simulink model "Demo_newformula"  (R2024b)
settings: Solver=FixedStepAuto  StartTime=0.0  StopTime=100  FixedStep=0.1  RelTol=1e-3
undefined symbols (not defined in the file or in its folder): LF
libraries: instrumentseriallib x4
settings Model: Creator=ihtis  LastModifiedBy=ihtisham

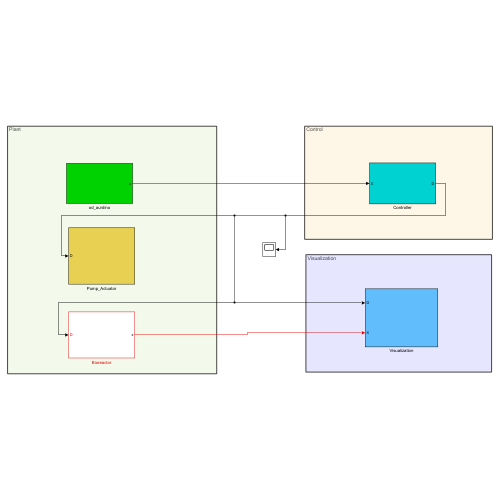
[thumbnail: Simulink's stored preview of the top-level diagram]
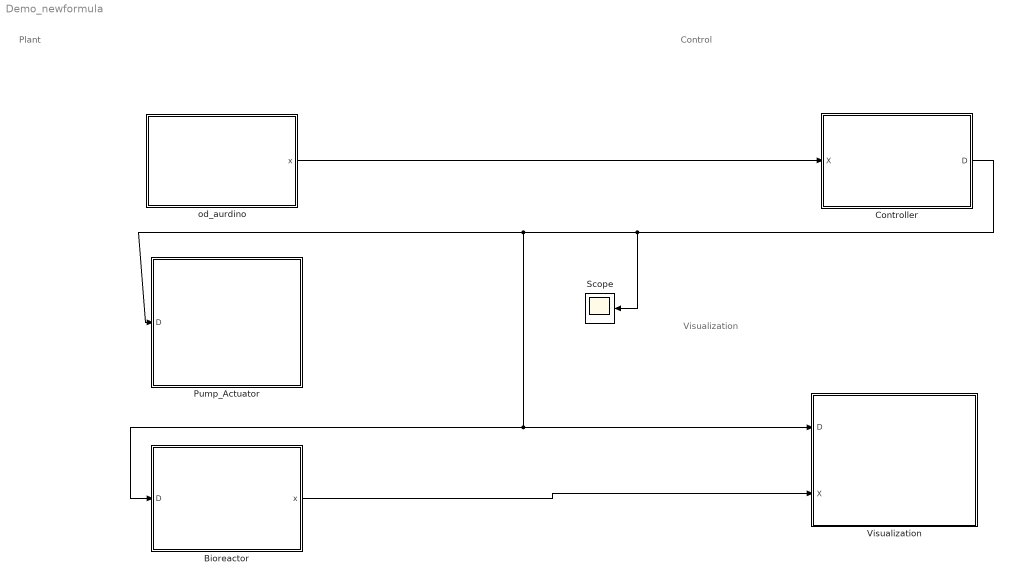
== system Demo_newformula ==
  note: Control
  note: Plant
  note: Visualization
  Bioreactor : Subsystem
  Controller : Subsystem
  Pump_Actuator : Subsystem
  Scope : Scope
  Visualization : Subsystem
  od_aurdino : Subsystem
  wires:
  Bioreactor/1(x) -> Visualization/2(X)
  Controller/1(D) -> Visualization/1(D), Bioreactor/1(D), Pump_Actuator/1(D), Scope/1
  od_aurdino/1(x) -> Controller/1(X)

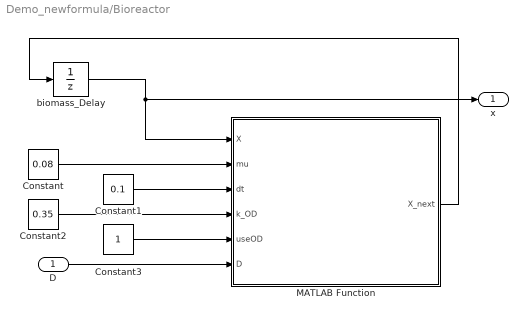
== system Demo_newformula/Bioreactor ==
  D : Inport
  Constant : Constant  Value=0.08
  Constant1 : Constant  Value=0.1
  Constant2 : Constant  Value=0.35
  Constant3 : Constant
  MATLAB Function : MATLAB Function  TreatAsAtomicUnit=on
  biomass_Delay : UnitDelay  InitialCondition=0.5  SampleTime=-1  HasFrameUpgradeWarning=on
  x : Outport
  wires:
  MATLAB Function/1(X_next) -> biomass_Delay/1
  Constant/1 -> MATLAB Function/2(mu)
  Constant1/1 -> MATLAB Function/3(dt)
  biomass_Delay/1 -> x/1, MATLAB Function/1(X)
  Constant2/1 -> MATLAB Function/4(k_OD)
  D/1 -> MATLAB Function/6(D)
  Constant3/1 -> MATLAB Function/5(useOD)

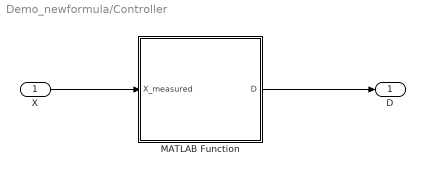
== system Demo_newformula/Controller ==
  X : Inport
  MATLAB Function : MATLAB Function  TreatAsAtomicUnit=on
  D : Outport
  wires:
  X/1 -> MATLAB Function/1(X_measured)
  MATLAB Function/1(D) -> D/1

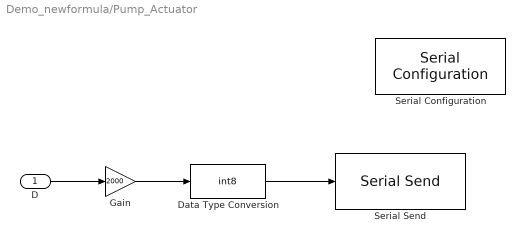
== system Demo_newformula/Pump_Actuator ==
  D : Inport
  Data Type Conversion : DataTypeConversion  OutDataTypeStr=int8  SaturateOnIntegerOverflow=off  RndMeth=Floor
  Gain : Gain  Gain=2000
  Serial Configuration : instrumentseriallib/Serial Configuration  Priority=-200000  PortSel=COM8  Port=COM8  ComPort=COM8  BaudRate=9600  DataBits=8  Parity=none  StopBits=1  ByteOrder=little-endian  FlowControl=none  Timeout=10  SimulateUsing=Interpreted execution  BlockInModel=on  aMode=1
      settings: LibrarySourceBlock=c2000lib/Host Communication/Serial Configuration
  Serial Send : instrumentseriallib/Serial Send  Priority=1  PortSel=COM8  Port=COM8  ComPort=COM8  Header=[]  Terminator=<none>  CustomTerminator=[]  EnableBlockingMode=on  SimulateUsing=Interpreted execution  BlockInModel=on  aMode=1
      settings: LibrarySourceBlock=c2000lib/Host Communication/Serial Send
  wires:
  D/1 -> Gain/1
  Gain/1 -> Data Type Conversion/1
  Data Type Conversion/1 -> Serial Send/1

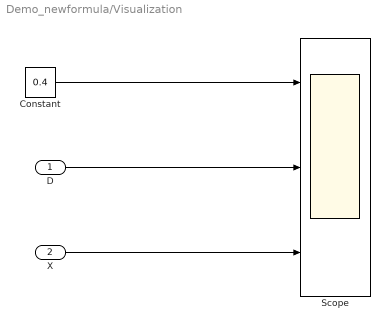
== system Demo_newformula/Visualization ==
  D : Inport
  X : Inport  Port=2
  Constant : Constant  Value=0.4
  Scope : Scope  NumInputPorts=3
  wires:
  X/1 -> Scope/3
  D/1 -> Scope/2
  Constant/1 -> Scope/1

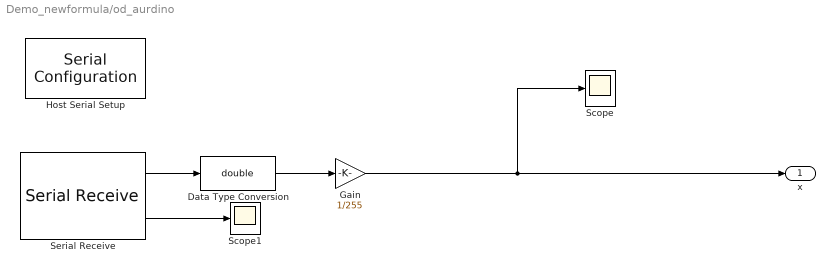
== system Demo_newformula/od_aurdino ==
  Data Type Conversion : DataTypeConversion  OutDataTypeStr=double  SaturateOnIntegerOverflow=off  RndMeth=Floor
  Gain : Gain  Gain=1/255
  Host Serial Setup : instrumentseriallib/Serial Configuration  Priority=-99  PortSel=COM5  Port=COM5  ComPort=COM5  BaudRate=9600  DataBits=8  Parity=none  StopBits=1  ByteOrder=little-endian  FlowControl=none  Timeout=2  SimulateUsing=Interpreted execution  BlockInModel=on  aMode=5
      settings: LibrarySourceBlock=mcblib/Protection and Diagnostics/Host Serial Setup
  Scope : Scope
  Scope1 : Scope
  Serial Receive : instrumentseriallib/Serial Receive  Priority=1  PortSel=COM5  Port=COM5  ComPort=COM5  DataType=uint8  SaveDataType=uint8  ToggleHeader=off  Header=[]  ToggleDataSize=on  DataSize=[1 1]  ToggleTerminator=off  Terminator=LF ('\n')  CustomTerminator=[]  InputFormat=Column major  EnableBlockingMode=off  ActionDataUnavailable=Output last received value  ActionWhenDataUnavailable=Output last received value  CustomValue=0  SampleTime=0.1  SimulateUsing=Interpreted execution  BlockInModel=on  aMode=1
      settings: LibrarySourceBlock=c2000lib/Host Communication/Serial Receive
  x : Outport
  wires:
  Serial Receive/1 -> Data Type Conversion/1
  Gain/1 -> Scope/1, x/1
  Serial Receive/2 -> Scope1/1
  Data Type Conversion/1 -> Gain/1

== matlab function Demo_newformula/Bioreactor/MATLAB Function ==
  data: X input; mu input; dt input; k_OD input; useOD input; X_next output; D input
function X_next = BiomassReactor(X, mu, dt, k_OD, useOD, D)
% Biomass or OD growth under exponential model with dilution

% Convert OD to biomass if needed
if useOD
    X_biomass = X * k_OD;
else
    X_biomass = X;
end

% Exponential growth + dilution
X_biomass_next = X_biomass + (mu - D) * X_biomass * dt;

% Avoid negative biomass
X_biomass_next = max(X_biomass_next, 0);

% Convert back to OD if required
if useOD
    X_next = X_biomass_next / k_OD;
else
    X_next = X_biomass_next;
end

== matlab function Demo_newformula/Controller/MATLAB Function ==
  data: X_measured input; D output
function D = Controller(X_measured)
persistent error_int
if isempty(error_int)
    error_int = 0;
end

% --- Controller parameters ---
OD_setpoint = 0.4;     % desired OD / biomass level
Kp = 0.25;             % proportional gain
Ki = 0.02;             % integral gain
dt = 0.1;              % same as simulation step time

% --- Compute control error ---
error = OD_setpoint - X_measured;

% --- Integrate error ---
error_int = error_int + error * dt;

% --- Compute control output (with correct sign for turbidostat) ---
D = 0.05 - (Kp * error + Ki * error_int);
%  ↑  note the minus sign (reduces D when OD < setpoint)

% --- Apply physical limits ---
D = max(min(D, 0.6), 0.01);   % between 0.01–0.5 1/h typical for algal dilution
end
